simulink model "Self_balance_robot_controller"  (R2025a)
settings: Solver=VariableStepAuto  StartTime=0.0  StopTime=5  RelTol=1e-3
values from neighbouring files (symbols this model uses):
  A22 = -B21_torque * k_v    (= -38.2602040566)    [lqr_controller.m]
  A23 = -(M^2 * l^2 * g) / Q_eq    (= -11.8742321134)    [lqr_controller.m]
  A42 = -B41_torque * k_v    (= 421.23380485)    [lqr_controller.m]
  A43 = (M * l * g * (M + 2 * m + (2 * I) / (r^2))) / Q_eq    (= 200.450238455)    [lqr_controller.m]
  B21 = B21_torque * k_u    (= 3.03833748845)    [lqr_controller.m]
  B41 = B41_torque * k_u    (= -33.4512188902)    [lqr_controller.m]
  Jeq = 0.0005    [JG25_370_Parmaters.m]    (also in lqr_controller.m)
  Ke_phi = 0.4092556    [JG25_370_Parmaters.m]    (also in lqr_controller.m)
  Km_phi = 0.1089611    [JG25_370_Parmaters.m]    (also in lqr_controller.m)
  La = 0.0005    [JG25_370_Parmaters.m]    (also in lqr_controller.m)
  Ra = 7.73798    [JG25_370_Parmaters.m]    (also in lqr_controller.m)
undefined symbols (not defined in the file or in its folder): K
settings Model: Creator=ASUS  LastModifiedBy=ASUS

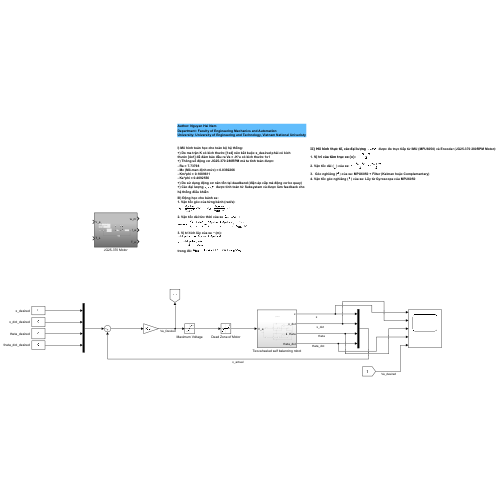
[thumbnail: Simulink's stored preview of the top-level diagram]
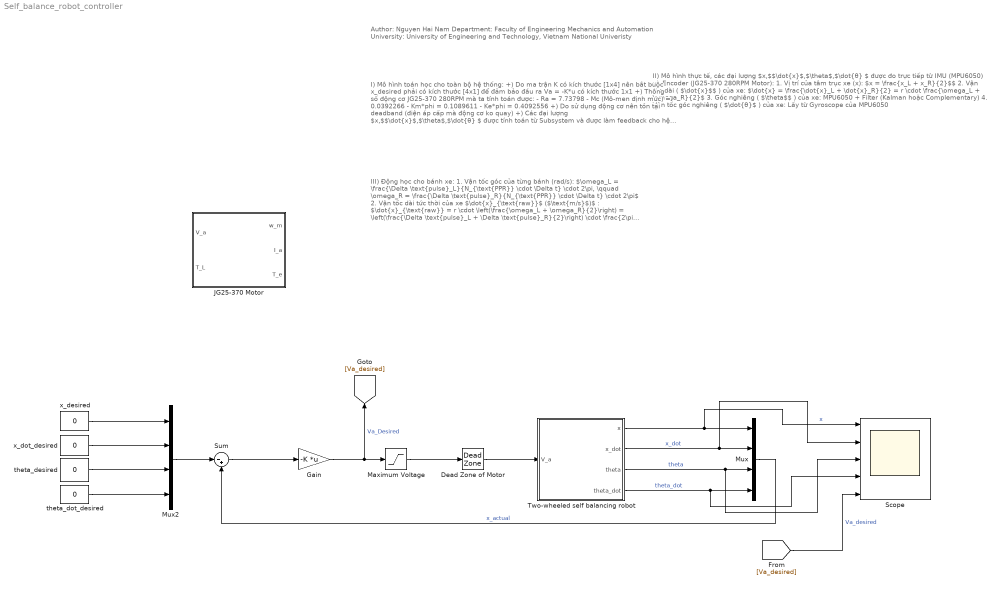
== system Self_balance_robot_controller ==
  note: Author: Nguyen Hai Nam
      | Department: Faculty of Engineering Mechanics and Automation
      | University: University of Engineering and Technology, Vietnam National Univeristy
  note: III) Động học cho bánh xe:
      | 1. Vận tốc góc của từng bánh (rad/s):
      | $\omega_L = \frac{\Delta \text{pulse}_L}{N_{\text{PPR}} \cdot \Delta t} \cdot 2\pi, \qquad \omega_R = \frac{\Delta \text{pulse}_R}{N_{\text{PPR}} \cdot \Delta t} \cdot 2\pi$
      | 2. Vận tốc dài tức thời của xe $\dot{x}_{\text{raw}}$ ($\text{m/s}$)$ :
      | $\dot{x}_{\text{raw}} = r \cdot \left(\frac{\omega_L + \omega_R}{2}\right) = \left(\frac{\Delta \text{pulse}_L + \Delta \text{pulse}_R}{2}\right) \cdot \frac{2\pi r}{N_{\text{PPR}} \cdot \Delta t}$$
      | 3. Vị trí tích lũy của xe $x$ (m):
      | $\text{total\_pulse} += (\Delta \text{pulse}_L + \Delta \text{pulse}_R)$$
      | $x = \frac{\text{total\_pulse}}{2} \cdot \frac{2\pi r}{N_{\text{PPR}}}$$
      | trong đó: $N_{\text{PPR}} = 11 \times 4 \times 21.3 = 937.2\text{ xung/vòng}$$
  note: II) Mô hình thực tế, các đại lượng $x,$$\dot{x}$,$\theta$,$\dot{θ} ​$ được đo trực tiếp từ IMU (MPU6050) và Encoder (JG25-370 280RPM Motor):
      | 1. Vị trí của tâm trục xe (x): $x = \frac{x_L + x_R}{2}$$
      | 2. Vận tốc dài ( $\dot{x}$$ ) của xe: $\dot{x} = \frac{\dot{x}_L + \dot{x}_R}{2} = r \cdot \frac{\omega_L + \omega_R}{2}$
      | 3. Góc nghiêng ( $\theta$$ ) của xe: MPU6050 + Filter (Kalman hoặc Complementary)
      | 4. Vận tốc góc nghiêng ( $\dot{θ}$ ) của xe: Lấy từ Gyroscope của MPU6050
  note: I) Mô hình toán học cho toàn bộ hệ thống:
      | +) Do ma trận K có kích thước [1x4] nên bắt buộc x_desired phải có kích
      | thước [4x1] để đảm bảo đầu ra Va = -K*u có kích thước 1x1
      | +) Thông số động cơ JG25-370 280RPM mà ta tính toán được:
      | - Ra = 7.73798
      | - Mc (Mô-men định mức) = 0.0392266
      | - Km*phi = 0.1089611
      | - Ke*phi = 0.4092556
      | +) Do sử dụng động cơ nên tồn tại deadband (điện áp cấp mà động cơ ko quay)
      | +) Các đại lượng $x,$$\dot{x}$,$\theta$,$\dot{θ} ​$ được tính toán từ Subsystem và được làm feedback cho
      | hệ thống điều khiển
  Dead Zone of Motor : DeadZone  LowerValue=-0.8  UpperValue=0.8
  Gain : Gain  Gain=-K  Multiplication=Matrix(K*u)
  JG25-370 Motor : Subsystem
  Maximum Voltage : Saturate  UpperLimit=12  LowerLimit=-12
  Mux : Mux
  Mux2 : Mux
  Scope : Scope  NumInputPorts=5
      settings: ActiveDisplayYMinimum=-0.12244644097582048  ActiveDisplayYMaximum=0.25591178971197603
  Sum : Sum  Inputs=|-+
  Two-wheeled self balancing robot : Subsystem
  theta_desired : Constant  Value=0
  theta_dot_desired : Constant  Value=0
  x_desired : Constant  Value=0
  x_dot_desired : Constant  Value=0
  wires:
  Two-wheeled self balancing robot/1(x) -> Scope/1, Mux/1  "x"
  Two-wheeled self balancing robot/2(x_dot) -> Scope/2, Mux/2  "x_dot"
  Two-wheeled self balancing robot/3(theta) -> Scope/3, Mux/3  "theta"
  Two-wheeled self balancing robot/4(theta_dot) -> Scope/4, Mux/4  "theta_dot"
  Mux2/1 -> Sum/1
  Sum/1 -> Gain/1
  Mux/1 -> Sum/2  "x_actual"
  x_desired/1 -> Mux2/1
  x_dot_desired/1 -> Mux2/2
  theta_dot_desired/1 -> Mux2/4
  theta_desired/1 -> Mux2/3
  Dead Zone of Motor/1 -> Two-wheeled self balancing robot/1(V_a)
  Maximum Voltage/1 -> Dead Zone of Motor/1
  Gain/1 -> Maximum Voltage/1, [Va_desired]  "Va_Desired"
  [Va_desired] -> Scope/5  "Va_desired"

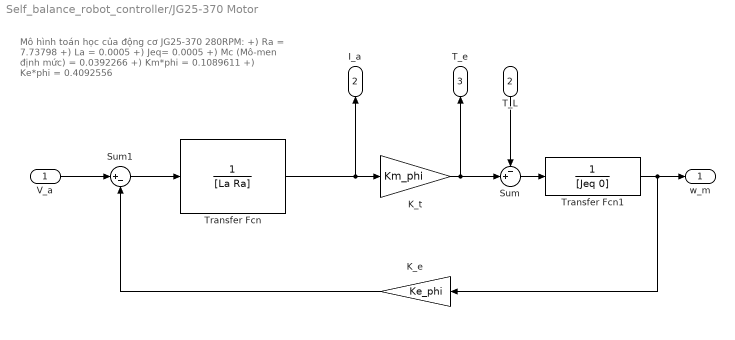
== system Self_balance_robot_controller/JG25-370 Motor ==
  note: Mô hình toán học của động cơ JG25-370 280RPM:
      | +) Ra = 7.73798
      | +) La = 0.0005
      | +) Jeq= 0.0005
      | +) Mc (Mô-men định mức) = 0.0392266
      | +) Km*phi = 0.1089611
      | +) Ke*phi = 0.4092556
  V_a : Inport
  T_L : Inport  Port=2
  K_e : Gain  Gain=Ke_phi
  K_t : Gain  Gain=Km_phi
  Sum : Sum  Inputs=-+|
  Sum1 : Sum  Inputs=|+-
  Transfer Fcn : TransferFcn  Denominator=[La Ra]
  Transfer Fcn1 : TransferFcn  Denominator=[Jeq 0]
  w_m : Outport
  I_a : Outport  Port=2
  T_e : Outport  Port=3
  wires:
  K_t/1 -> T_e/1, Sum/2
  Sum/1 -> Transfer Fcn1/1
  Transfer Fcn1/1 -> w_m/1, K_e/1
  Sum1/1 -> Transfer Fcn/1
  V_a/1 -> Sum1/1
  K_e/1 -> Sum1/2
  Transfer Fcn/1 -> I_a/1, K_t/1
  T_L/1 -> Sum/1

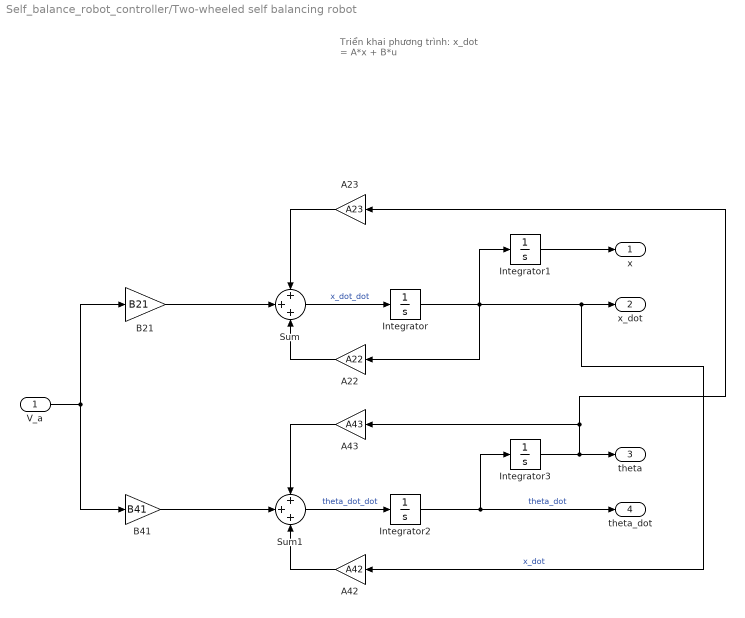
== system Self_balance_robot_controller/Two-wheeled self balancing robot ==
  note: Triển khai phương trình:
      | x_dot = A*x + B*u
  V_a : Inport
  A22 : Gain  Gain=A22
  A23 : Gain  Gain=A23
  A42 : Gain  Gain=A42
  A43 : Gain  Gain=A43
  B21 : Gain  Gain=B21
  B41 : Gain  Gain=B41
  Integrator : Integrator
  Integrator1 : Integrator  InitialCondition=0.2
  Integrator2 : Integrator
  Integrator3 : Integrator  InitialCondition=0.1
  Sum : Sum  Inputs=+++
  Sum1 : Sum  Inputs=+++
  x : Outport
  x_dot : Outport  Port=2
  theta : Outport  Port=3
  theta_dot : Outport  Port=4
  wires:
  A23/1 -> Sum/1
  B21/1 -> Sum/2
  V_a/1 -> B21/1, B41/1
  A22/1 -> Sum/3
  Sum/1 -> Integrator/1  "x_dot_dot"
  Integrator/1 -> A22/1, Integrator1/1, x_dot/1, A42/1  "x_dot"
  Integrator1/1 -> x/1
  B41/1 -> Sum1/2
  A43/1 -> Sum1/1
  Sum1/1 -> Integrator2/1  "theta_dot_dot"
  Integrator2/1 -> theta_dot/1, Integrator3/1  "theta_dot"
  Integrator3/1 -> theta/1, A23/1, A43/1
  A42/1 -> Sum1/3
